simulink model "homeMobileManipulator"  (R2026a)
settings: Solver=ode4  StartTime=0  StopTime=Inf  FixedStep=cfg.rates.plant  MaxStep=cfg.rates.plant  AbsTol=1e-8
PostLoadFcn:
  | hmmSetup;
InitFcn:
  | hmmInitializeRun(bdroot);
values from neighbouring files (symbols this model uses):
  armJointLimits = zeros(numel(idx.arm), 2)    [hmmSetup.m]
  cfg = app.RunCfg    [HomeMobileManipulatorApp.m]    (also in HomeMobileManipulatorExample.m = params.cfg; hmmSetup.m = hmmConfig(); setupParams.m = data.cfg)
undefined symbols (not defined in the file or in its folder): actionQueueInit, actorNameTable, Angle, apertureMap, armPlanInit, Axis, basePlanInit, Custom, Extent, gray, gripperCoupling, invalidRayHits, movableRegistry, objectTargetInit, perceptionStatusInit, placeTargetInit, Position, robotStateInit, Sim3dSensor
libraries: robotmaniplib x20, robotcorelib x18, simulink x9, sim3dcameralib x6, sim3dgroundtruthsensorlib x4, dspmtrx3 x3, slpidlib x3, sim3dlib x3, hdlsllib x2, robotsim3dlib x1
(part 1 of 6)
PreSaveFcn:
  | if exist('hmmCleanBeforeSave', 'file'), hmmCleanBeforeSave(bdroot); end
settings Model: SimulationMode=accelerator  Creator=rvalenti  LastModifiedBy=rvalenti

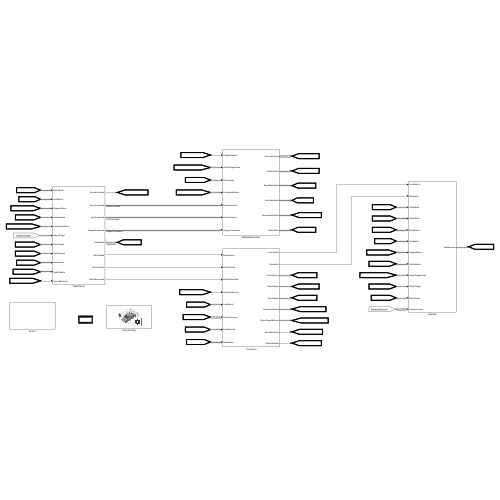
[thumbnail: Simulink's stored preview of the top-level diagram]
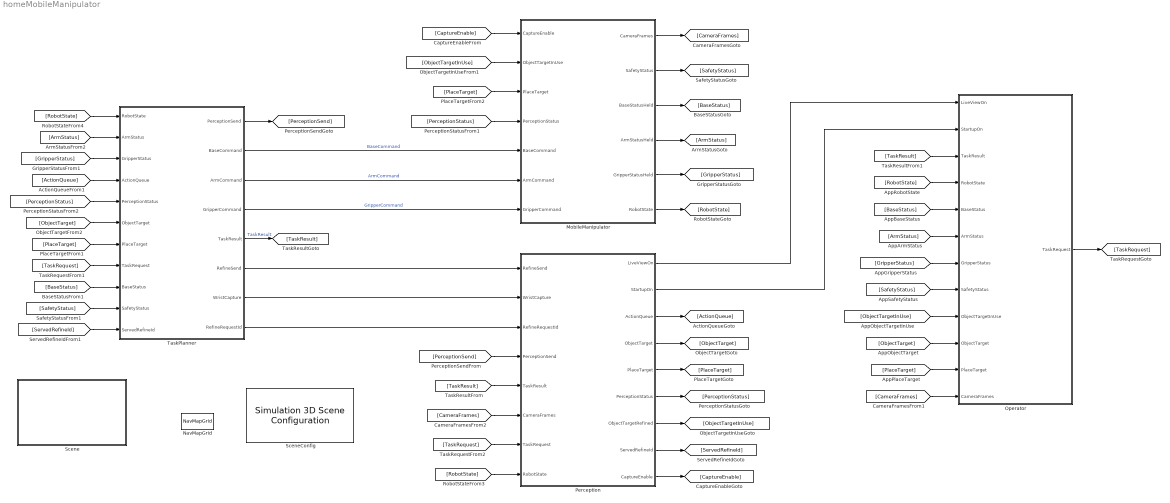
== system homeMobileManipulator ==
  MobileManipulator : Subsystem
  NavMapGrid : DataStoreMemory  DataStoreName=NavMapGrid  InitialValue=navMapGrid  ShowAdditionalParam=off
      settings: DataLoggingMaxPoints=5
  Operator : Subsystem
  Perception : Subsystem
  Scene : Subsystem
  SceneConfig : sim3dlib/Simulation 3D Scene Configuration  Priority=0  ProjectFormat=Default Scenes  SceneDesc=Empty scene  ProjectName=C:\Program Files\MATLAB\R2026a\toolbox\shared\sim3d_projects\automotive_project_windows\UE\WindowsNoEditor\VehicleSimulation.exe  ScenePath=/Game/Maps/EmptyScene  EnableOpenDRIVE=off  vehTagList={'<empty>';'Custom';'Scene Origin';'Sim3dActor1';'Sim3dActor2';'SimulinkVehicle1'}  vehTag=Scene Origin  AttachedCameraRelativeTranslation=[0 0 0]  FreeCameraDefaultInitialTranslation=cfg.view.translation  AttachedCameraRelativeRotation=[0, -15, 0]  FreeCameraDefaultInitialRotation=cfg.view.rotationDeg  ViewpointName=Custom  parentTag=HomeMobileManipulator  FreeCameraInitialTranslation=[0 0 0]  FreeCameraInitialRotation=[0 0 0]  OpVisEn=off  Ts=cfg.rates.scene  EnableWindow=on  EnableRemoteAccess=off  SimulationMode=CoSimulation  SimulateUsing=Interpreted execution  EnableAnimationRecording=off  OverrideDefaultRecording=off  AnimationRecordingFileName=sim3dAnimation.mat  AnimationRecordingInterval=[0 inf]  EnableWeather=off  SunAzimuth=sunAzimuth  SunAltitude=sunAltitude  EnableGeospatialSun=off  Latitude=0  Longitude=0  Date=2023-01-01  Time=10:30:00  GeoTimeZone=-5.0  SunDaylightSaving=off  wind=1  clouds=10  EnableVolumetricClouds=off  CloudCoverage=0  CloudAltitude=6  fog=0  rain=0  RaindropsEffect=off  SnowDensity=0  EnableGeospatial=off  TilesetSource=Earth terrain  UseTrueOrigin=off  OriginHeight=200  OriginLatitude=40.744652  OriginLongitude=-73.988864  MapStyle=Aerial  AdditionalAssetIDs=[]  UseAdvancedSunSky=off  SolarTime=11  TimeZone=-5  Day=21  Month=9  Year=2022  UseDaylightSavingTime=on  DSTStartDay=10  DSTStartMonth=3  DSTEndDay=3  DSTEndMonth=11  DSTSwitchHour=2  sensorTag=MainCamera3  sensorId=3  sensorName=MainCamera3  mountLoc=Origin  offsetFlag=off  tmountOffset=[0, 0, 0]  rmountOffset=[0, 0, 0]  HorizontalResolution=1280  VerticalResolution=720  HorizontalFOV=cfg.view.hfovDeg  mountPoint=[0 0 0]  mountOrientation=[0 0 0]  aMode=5  ID=3  GeoTrigger=Inactive  ViewNameList={'Custom'}  ViewTranslationList={'[0 0 0]'}  ViewRotationList={'[0 0 0]'}
      settings: LibrarySourceBlock=sl3dlib/Simulation 3D/Environment/Simulation 3D Scene Configuration
  TaskPlanner : Subsystem
  wires:
  [TaskRequest] -> TaskPlanner/8(TaskRequest)
  [RobotState] -> TaskPlanner/1(RobotState)
  [ObjectTarget] -> TaskPlanner/6(ObjectTarget)
  [SafetyStatus] -> TaskPlanner/10(SafetyStatus)
  TaskPlanner/5(TaskResult) -> [TaskResult]  "TaskResult"
  [BaseStatus] -> TaskPlanner/9(BaseStatus)
  [ArmStatus] -> TaskPlanner/2(ArmStatus)
  [GripperStatus] -> TaskPlanner/3(GripperStatus)
  [PerceptionStatus] -> TaskPlanner/5(PerceptionStatus)
  [PlaceTarget] -> TaskPlanner/7(PlaceTarget)
  [ActionQueue] -> TaskPlanner/4(ActionQueue)
  [ServedRefineId] -> TaskPlanner/11(ServedRefineId)
  TaskPlanner/2(BaseCommand) -> MobileManipulator/5(BaseCommand)  "BaseCommand"
  TaskPlanner/3(ArmCommand) -> MobileManipulator/6(ArmCommand)  "ArmCommand"
  [ObjectTargetInUse] -> MobileManipulator/2(ObjectTargetInUse)
  [PlaceTarget] -> MobileManipulator/3(PlaceTarget)
  TaskPlanner/4(GripperCommand) -> MobileManipulator/7(GripperCommand)  "GripperCommand"
  MobileManipulator/1(CameraFrames) -> [CameraFrames]
  [PerceptionStatus] -> MobileManipulator/4(PerceptionStatus)
  MobileManipulator/2(SafetyStatus) -> [SafetyStatus]
  MobileManipulator/3(BaseStatusHeld) -> [BaseStatus]
  MobileManipulator/4(ArmStatusHeld) -> [ArmStatus]
  MobileManipulator/5(GripperStatusHeld) -> [GripperStatus]
  MobileManipulator/6(RobotState) -> [RobotState]
  [CameraFrames] -> Perception/6(CameraFrames)
  [TaskRequest] -> Perception/7(TaskRequest)
  [RobotState] -> Perception/8(RobotState)
  Perception/3(ActionQueue) -> [ActionQueue]
  Perception/4(ObjectTarget) -> [ObjectTarget]
  Perception/5(PlaceTarget) -> [PlaceTarget]
  Perception/6(PerceptionStatus) -> [PerceptionStatus]
  TaskPlanner/7(WristCapture) -> Perception/2(WristCapture)
  Perception/9(CaptureEnable) -> [CaptureEnable]
  TaskPlanner/8(RefineRequestId) -> Perception/3(RefineRequestId)
  Perception/7(ObjectTargetRefined) -> [ObjectTargetInUse]
  TaskPlanner/1(PerceptionSend) -> [PerceptionSend]
  TaskPlanner/6(RefineSend) -> Perception/1(RefineSend)
  Perception/8(ServedRefineId) -> [ServedRefineId]
  Operator/1(TaskRequest) -> [TaskRequest]
  [RobotState] -> Operator/4(RobotState)
  [BaseStatus] -> Operator/5(BaseStatus)
  [ArmStatus] -> Operator/6(ArmStatus)
  [GripperStatus] -> Operator/7(GripperStatus)
  [SafetyStatus] -> Operator/8(SafetyStatus)
  [ObjectTargetInUse] -> Operator/9(ObjectTargetInUse)
  [ObjectTarget] -> Operator/10(ObjectTarget)
  [PlaceTarget] -> Operator/11(PlaceTarget)
  [CameraFrames] -> Operator/12(CameraFrames)
  Perception/1(LiveViewOn) -> Operator/1(LiveViewOn)
  Perception/2(StartupOn) -> Operator/2(StartupOn)
  [PerceptionSend] -> Perception/4(PerceptionSend)
  [TaskResult] -> Perception/5(TaskResult)
  [TaskResult] -> Operator/3(TaskResult)
  [CaptureEnable] -> MobileManipulator/1(CaptureEnable)

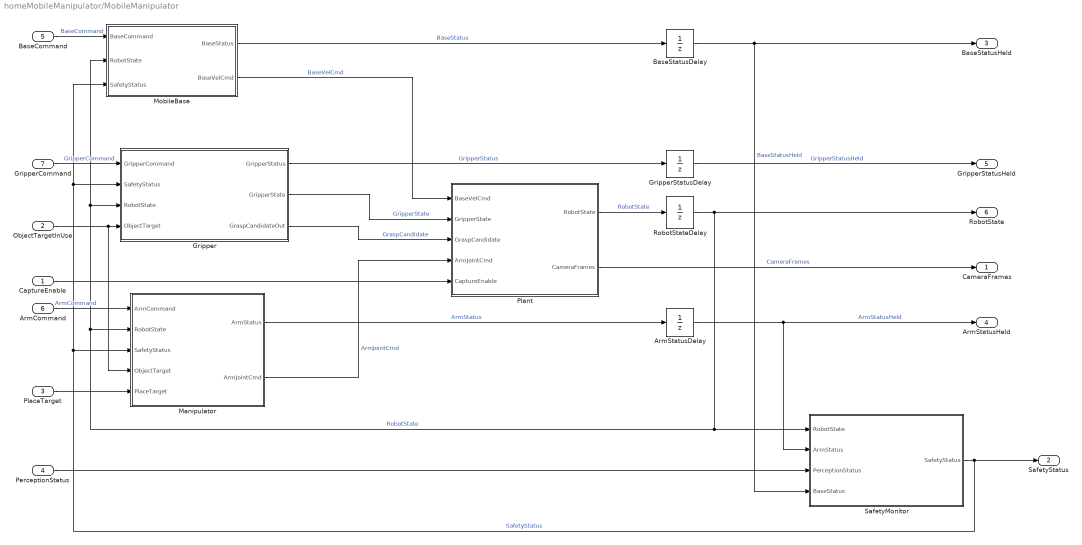
== system homeMobileManipulator/MobileManipulator ==
  CaptureEnable : Inport
  ObjectTargetInUse : Inport  Port=2
  PlaceTarget : Inport  Port=3
  PerceptionStatus : Inport  Port=4
  BaseCommand : Inport  Port=5
  ArmCommand : Inport  Port=6
  GripperCommand : Inport  Port=7
  ArmStatusDelay : UnitDelay  SampleTime=cfg.rates.supervisor
  BaseStatusDelay : UnitDelay  SampleTime=cfg.rates.supervisor
  Gripper : Subsystem
  GripperStatusDelay : UnitDelay  SampleTime=cfg.rates.supervisor
  Manipulator : Subsystem
  MobileBase : Subsystem
  Plant : Subsystem
  RobotStateDelay : UnitDelay  Description=|  InitialCondition=robotStateInit  SampleTime=cfg.rates.plant
      | Breaks the plant-to-supervisor algebraic loop: the supervisors read the robot state and the plant reads their commands, so one of the two has to see the previous step.
      | 
      | THE INITIAL CONDITION IS THE ROBOT'S TRUE STARTING STATE, NOT A ZEROED BUS, AND THAT IS LOAD-BEARING. On the first step every consumer sees this value instead of a measurement. Zeroed, ArmJointPos is the UR5e's fully outstretched pose - tool 1.11 m from arm_mount against a cfg.arm.reach of 0.85 - so SafetyMonitor's reach check fired on sample 0, the e-stop latched, and all four charts sat in their terminal stopped mode for the whole run. hmmSetup builds robotStateInit from cfg.base.initialPose and cfg.arm.stowConfig, the same values the plant's integrators start from, and measures the tool pose off the assembled tree so it cannot drift from the plant's kinematics.
  SafetyMonitor : Subsystem  Description=|  TreatAsAtomicUnit=on  SystemSampleTime=cfg.rates.control
      | Independent limit monitor and the single source of the latched e-stop.
      | 
      | It reads only measured state and reported status - never a chart internal - so a supervisor that has lost track of itself cannot suppress its own e-stop. Every limit is re-evaluated every step; the latch is what makes the result terminal. EStop reaches all four charts (TaskPlanner, BaseSupervisor, ArmSupervisor, GripperSupervisor) through one root Unit Delay, and each has a defined safe terminal mode for it.
      | 
      | ClearanceThreshold is published on the bus rather than assumed, so the value the monitor compared against can be audited against the margin the planner used. hmmSetup/assertConfigInvariants errors at load if the two ever diverge.
  CameraFrames : Outport
  SafetyStatus : Outport  Port=2
  BaseStatusHeld : Outport  Port=3
  ArmStatusHeld : Outport  Port=4
  GripperStatusHeld : Outport  Port=5
  RobotState : Outport  Port=6
  wires:
  BaseStatusDelay/1 -> BaseStatusHeld/1, SafetyMonitor/4(BaseStatus)  "BaseStatusHeld"
  PerceptionStatus/1 -> SafetyMonitor/3(PerceptionStatus)
  Manipulator/2(ArmJointCmd) -> Plant/4(ArmJointCmd)  "ArmJointCmd"
  BaseCommand/1 -> MobileBase/1(BaseCommand)  "BaseCommand"
  GripperCommand/1 -> Gripper/1(GripperCommand)  "GripperCommand"
  ArmCommand/1 -> Manipulator/1(ArmCommand)  "ArmCommand"
  ObjectTargetInUse/1 -> Gripper/4(ObjectTarget), Manipulator/4(ObjectTarget)
  PlaceTarget/1 -> Manipulator/5(PlaceTarget)
  Gripper/1(GripperStatus) -> GripperStatusDelay/1  "GripperStatus"
  Gripper/2(GripperState) -> Plant/2(GripperState)  "GripperState"
  Gripper/3(GraspCandidateOut) -> Plant/3(GraspCandidate)  "GraspCandidate"
  Manipulator/1(ArmStatus) -> ArmStatusDelay/1  "ArmStatus"
  MobileBase/2(BaseVelCmd) -> Plant/1(BaseVelCmd)  "BaseVelCmd"
  MobileBase/1(BaseStatus) -> BaseStatusDelay/1  "BaseStatus"
  CaptureEnable/1 -> Plant/5(CaptureEnable)
  GripperStatusDelay/1 -> GripperStatusHeld/1  "GripperStatusHeld"
  ArmStatusDelay/1 -> ArmStatusHeld/1, SafetyMonitor/2(ArmStatus)  "ArmStatusHeld"
  Plant/1(RobotState) -> RobotStateDelay/1  "RobotState"
  Plant/2(CameraFrames) -> CameraFrames/1  "CameraFrames"
  RobotStateDelay/1 -> RobotState/1, MobileBase/2(RobotState), Gripper/3(RobotState), Manipulator/2(RobotState), SafetyMonitor/1(RobotState)  "RobotState"
  SafetyMonitor/1(SafetyStatus) -> MobileBase/3(SafetyStatus), Gripper/2(SafetyStatus), Manipulator/3(SafetyStatus), SafetyStatus/1  "SafetyStatus"

== system homeMobileManipulator/Operator ==
  LiveViewOn : Inport
  StartupOn : Inport  Port=2
  TaskResult : Inport  Port=3
  RobotState : Inport  Port=4
  BaseStatus : Inport  Port=5
  ArmStatus : Inport  Port=6
  GripperStatus : Inport  Port=7
  SafetyStatus : Inport  Port=8
  ObjectTargetInUse : Inport  Port=9
  ObjectTarget : Inport  Port=10
  PlaceTarget : Inport  Port=11
  CameraFrames : Inport  Port=12
  AppStateTap : MATLAB Function  TreatAsAtomicUnit=on  SystemSampleTime=0.2
  LiveViewTap : MATLAB Function  TreatAsAtomicUnit=on  SystemSampleTime=cfg.rates.perception
  LiveViewTapOpen : Terminator
  TaskRequestSource : MATLAB Function  TreatAsAtomicUnit=on
  TaskRequest : Outport
  wires:
  CameraFrames/1 -> LiveViewTap/1(CameraFrames)
  LiveViewOn/1 -> LiveViewTap/2(LiveViewOn)
  PlaceTarget/1 -> AppStateTap/9(PlaceTarget)
  BaseStatus/1 -> AppStateTap/3(BaseStatus)
  TaskResult/1 -> AppStateTap/2(TaskResult)  "TaskResult"
  StartupOn/1 -> LiveViewTap/3(StartupOn)
  RobotState/1 -> AppStateTap/1(RobotState)
  GripperStatus/1 -> AppStateTap/5(GripperStatus)
  ArmStatus/1 -> AppStateTap/4(ArmStatus)
  SafetyStatus/1 -> AppStateTap/6(SafetyStatus)
  ObjectTargetInUse/1 -> AppStateTap/7(ObjectTargetRefined)
  ObjectTarget/1 -> AppStateTap/8(ObjectTarget)
  TaskRequestSource/1(task) -> TaskRequest/1
  LiveViewTap/1(Fired) -> LiveViewTapOpen/1

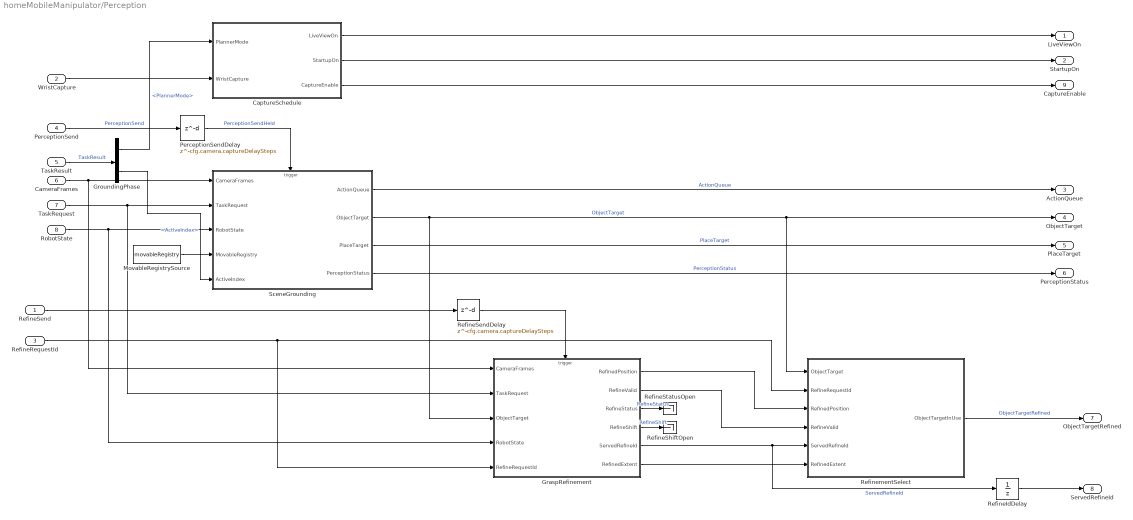
== system homeMobileManipulator/Perception ==
  RefineSend : Inport
  WristCapture : Inport  Port=2
  RefineRequestId : Inport  Port=3
  PerceptionSend : Inport  Port=4
  TaskResult : Inport  Port=5
  CameraFrames : Inport  Port=6
  TaskRequest : Inport  Port=7
  RobotState : Inport  Port=8
  CaptureSchedule : Subsystem
  GraspRefinement : Subsystem
  GroundingPhase : BusSelector  OutputSignals=PlannerMode,ActiveIndex
  MovableRegistrySource : Constant  Value=movableRegistry  OutDataTypeStr=Bus: MovableRegistry  SampleTime=cfg.rates.control
  PerceptionSendDelay : Delay  Description=|  DelayLength=cfg.camera.captureDelaySteps  InitialCondition=0  SampleTime=cfg.rates.supervisor
      | A DELAY OF cfg.camera.captureWindow, NOT A UNIT DELAY, and the length is the whole point. It still breaks the loop from Perception through the planner and back to Perception's trigger, which is why a delay is here at all.
      | 
      | The extra length exists because Plant/CameraRig is now gated on the grounding phase. The planner enters Grounding on a supervisor tick (0.02 s) and the rig captures on a perception tick (0.1 s). With a one-step delay the trigger would fire 0.02 s after the gate opened, before the rig had run, and Perception would read a held frame with Valid = false - or, on a second task, the frame from the first one. Holding the trigger back by three perception periods puts whole capture ticks between the gate opening and Perception looking.
      | 
      | The cost is that every task starts 0.30 s later than it used to. cfg.sup.timeout.ground is 22 s, so the phase has room for it.
      | 
      | See cfg.camera.captureWindow.
  RefineIdDelay : UnitDelay  SampleTime=-1
  RefineSendDelay : Delay  DelayLength=cfg.camera.captureDelaySteps
  RefineShiftOpen : Terminator
  RefineStatusOpen : Terminator
  RefinementSelect : Subsystem
  SceneGrounding : Subsystem
  LiveViewOn : Outport
  StartupOn : Outport  Port=2
  ActionQueue : Outport  Port=3
  ObjectTarget : Outport  Port=4
  PlaceTarget : Outport  Port=5
  PerceptionStatus : Outport  Port=6
  ObjectTargetRefined : Outport  Port=7
  ServedRefineId : Outport  Port=8
  CaptureEnable : Outport  Port=9
  wires:
  PerceptionSend/1 -> PerceptionSendDelay/1  "PerceptionSend"
  GroundingPhase/1 -> CaptureSchedule/1(PlannerMode)  "<PlannerMode>"
  WristCapture/1 -> CaptureSchedule/2(WristCapture)
  CameraFrames/1 -> SceneGrounding/1(CameraFrames), GraspRefinement/1(CameraFrames)
  TaskResult/1 -> GroundingPhase/1  "TaskResult"
  PerceptionSendDelay/1 -> SceneGrounding/Trigger  "PerceptionSendHeld"
  GroundingPhase/2 -> SceneGrounding/5(ActiveIndex)  "<ActiveIndex>"
  MovableRegistrySource/1 -> SceneGrounding/4(MovableRegistry)
  TaskRequest/1 -> SceneGrounding/2(TaskRequest), GraspRefinement/2(TaskRequest)
  RobotState/1 -> SceneGrounding/3(RobotState), GraspRefinement/4(RobotState)
  CaptureSchedule/1(LiveViewOn) -> LiveViewOn/1
  RefineSend/1 -> RefineSendDelay/1
  CaptureSchedule/2(StartupOn) -> StartupOn/1
  CaptureSchedule/3(CaptureEnable) -> CaptureEnable/1
  SceneGrounding/1(ActionQueue) -> ActionQueue/1  "ActionQueue"
  SceneGrounding/2(ObjectTarget) -> ObjectTarget/1, RefinementSelect/1(ObjectTarget), GraspRefinement/3(ObjectTarget)  "ObjectTarget"
  SceneGrounding/3(PlaceTarget) -> PlaceTarget/1  "PlaceTarget"
  SceneGrounding/4(PerceptionStatus) -> PerceptionStatus/1  "PerceptionStatus"
  RefineSendDelay/1 -> GraspRefinement/Trigger
  RefineRequestId/1 -> GraspRefinement/5(RefineRequestId), RefinementSelect/2(RefineRequestId)
  GraspRefinement/1(RefinedPosition) -> RefinementSelect/3(RefinedPosition)
  GraspRefinement/2(RefineValid) -> RefinementSelect/4(RefineValid)
  GraspRefinement/3(RefineStatus) -> RefineStatusOpen/1  "RefineStatus"
  GraspRefinement/4(RefineShift) -> RefineShiftOpen/1  "RefineShift"
  GraspRefinement/5(ServedRefineId) -> RefinementSelect/5(ServedRefineId), RefineIdDelay/1  "ServedRefineId"
  GraspRefinement/6(RefinedExtent) -> RefinementSelect/6(RefinedExtent)
  RefinementSelect/1(ObjectTargetInUse) -> ObjectTargetRefined/1  "ObjectTargetRefined"
  RefineIdDelay/1 -> ServedRefineId/1

== system homeMobileManipulator/Scene ==
  ApartmentShell : sim3dlib/Simulation 3D Actor  Priority=1  ActorName=Sim3dActor1  ParentName=Scene Origin  Operation=Create at setup  InitScriptText=|  SampleTime=-1  Translation=[0 0 0]  Rotation=[0 0 0]  Scale=[1 1 1]  aMode=aMode  ActorTag=Sim3dActor1  ActorType=Sim3dActor  ID=1
      | % Static apartment shell. The mesh is DISCOVERED at init time, never named by
      | % an absolute path in this block, so the model is portable between machines.
      | hmmLoadSceneShell(Actor);
  PropsStatusOpen : Terminator
  SceneProps : sim3dlib/Simulation 3D Actor  Priority=1  ActorName=Sim3dActor2  ParentName=Scene Origin  Operation=Create at setup  InitScriptText=|  SampleTime=-1  Translation=[0 0 0]  Rotation=[0 0 0]  Scale=[1 1 1]  aMode=aMode  ActorTag=Sim3dActor2  ActorType=Sim3dActor  ID=2
      | % Every movable prop the scene manifest lists, spawned as CHILDREN of this
      | % actor. ONE block spawns all of them on purpose: a block per prop would put
      | % the scene's contents into the model, which is the task-specific datum
      | % the design forbids. This actor itself carries no geometry and no transform -
      | % it exists to own the init script and to be the parent, which leaves manifest
      | % coordinates as world coordinates.
      | %
      | % THE PARENT IS NOT DECORATION. Props added at the world root from a block init
      | % script are accepted by the world and never reach the renderer, which is why
      | % this scene had furniture and nothing on it.
      | hmmSpawnProps(World, Actor);
  ShellStatusOpen : Terminator
  wires:
  SceneProps/1 -> PropsStatusOpen/1
  ApartmentShell/1 -> ShellStatusOpen/1

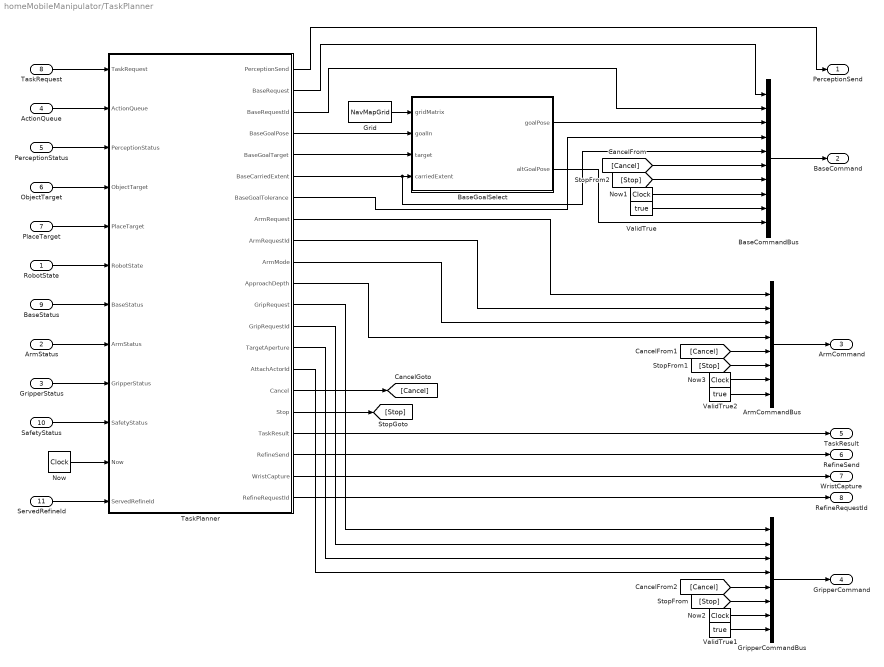
== system homeMobileManipulator/TaskPlanner ==
  RobotState : Inport  OutDataTypeStr=Bus: RobotState
  ArmStatus : Inport  Port=2  OutDataTypeStr=Bus: ArmStatus
  GripperStatus : Inport  Port=3  OutDataTypeStr=Bus: GripperStatus
  ActionQueue : Inport  Port=4  OutDataTypeStr=Bus: ActionQueue
  PerceptionStatus : Inport  Port=5  OutDataTypeStr=Bus: PerceptionStatus
  ObjectTarget : Inport  Port=6  OutDataTypeStr=Bus: ObjectTarget
  PlaceTarget : Inport  Port=7  OutDataTypeStr=Bus: PlaceTarget
  TaskRequest : Inport  Port=8  OutDataTypeStr=Bus: TaskRequest
  BaseStatus : Inport  Port=9  OutDataTypeStr=Bus: BaseStatus
  SafetyStatus : Inport  Port=10  OutDataTypeStr=Bus: SafetyStatus
  ServedRefineId : Inport  Port=11
  ArmCommandBus : BusCreator  Inputs=8  OutDataTypeStr=Bus: ArmCommand
      settings: InheritFromInputs=off
  BaseCommandBus : BusCreator  Inputs=10  OutDataTypeStr=Bus: BaseCommand
      settings: InheritFromInputs=off
  BaseGoalSelect : MATLAB Function  TreatAsAtomicUnit=on
  Grid : DataStoreRead  DataStoreName=NavMapGrid  SampleTime=cfg.rates.supervisor  IndexOptions=Index vector (dialog)  Indices=1  OutputSizes=1
  GripperCommandBus : BusCreator  Inputs=8  OutDataTypeStr=Bus: GripperCommand
      settings: InheritFromInputs=off
  Now{,1..3} (4 alike) : DigitalClock  SampleTime=cfg.rates.supervisor
  TaskPlanner : Stateflow chart  TreatAsAtomicUnit=on
      settings: PortSchema="{\"entries\":[{\"content\":{\"sides\":[{\"content\":{\"connectorIds\":[\"In1\",\"In2\",\"In3\",\"In4\",\"In5\",\"In6\",\"In7\",\"In8\",\"In9\",\"In10\",\"In11\",\"In12\"]},\"type\":\"ConnectorPlacement.EquallySpacedRectSide\",\"uuid\":\"f5e67e83-1d8e-420a-969a-b33278afb01c\"},{\"content\":{\"connectorIds\":[\"Out1\",\"Out2\",\"Out3\",\"Out4\",\"Out5\",\"Out7\",\"Out6\",\"Out8\",\"Out9\",\"Out10\",\"Out11\",\"Out12\",\"Out13\",\"Out14\",\"Out15\",\"Out16\",\"Out17\",\"Out18\",\"Out19\",\"Out20\",\"Out21\"],\"side\":\"RIGHT\"},\"type\":\"ConnectorPlacement.EquallySpacedRectSide\",\"uuid\":\"27a68318-2a47-4f3a-bcd2-e12b0ee86ade\"},{\"content\":{\"side\":\"TOP\"},\"type\":\"ConnectorPlacement.EquallySpacedRectSide\",\"uuid\":\"c7e5a260-d40c-4877-a934-6fb5002bb041\"}]},\"type\":\"ConnectorPlacement.EquallySpacedConnector\",\"uuid\":\"a1ee6b7c-e063-49c8-8f03-48fb3b9dd891\"}],\"packageUris\":[\"http://schema.mathworks.com/mf0/Connector/R2020b\"],\"version\":\"1.0\"}"
  ValidTrue : Constant  Value=true  OutDataTypeStr=boolean
  ValidTrue1 : Constant  Value=true  OutDataTypeStr=boolean
  ValidTrue2 : Constant  Value=true  OutDataTypeStr=boolean
  PerceptionSend : Outport
  BaseCommand : Outport  Port=2  OutDataTypeStr=Bus: BaseCommand
  ArmCommand : Outport  Port=3  OutDataTypeStr=Bus: ArmCommand
  GripperCommand : Outport  Port=4  OutDataTypeStr=Bus: GripperCommand
  TaskResult : Outport  Port=5  OutDataTypeStr=Bus: TaskResult
  RefineSend : Outport  Port=6
  WristCapture : Outport  Port=7
  RefineRequestId : Outport  Port=8
  wires:
  TaskPlanner/19(RefineSend) -> RefineSend/1
  TaskRequest/1 -> TaskPlanner/1(TaskRequest)
  BaseStatus/1 -> TaskPlanner/7(BaseStatus)
  PerceptionStatus/1 -> TaskPlanner/3(PerceptionStatus)
  ActionQueue/1 -> TaskPlanner/2(ActionQueue)
  ObjectTarget/1 -> TaskPlanner/4(ObjectTarget)
  Grid/1 -> BaseGoalSelect/1(gridMatrix)
  PlaceTarget/1 -> TaskPlanner/5(PlaceTarget)
  RobotState/1 -> TaskPlanner/6(RobotState)
  ArmStatus/1 -> TaskPlanner/8(ArmStatus)
  TaskPlanner/6(BaseGoalTolerance) -> BaseCommandBus/4
  GripperStatus/1 -> TaskPlanner/9(GripperStatus)
  TaskPlanner/15(AttachActorId) -> GripperCommandBus/4
  ServedRefineId/1 -> TaskPlanner/12(ServedRefineId)
  SafetyStatus/1 -> TaskPlanner/10(SafetyStatus)
  Now2/1 -> GripperCommandBus/7
  TaskPlanner/13(GripRequestId) -> GripperCommandBus/2
  Now/1 -> TaskPlanner/11(Now)
  TaskPlanner/3(BaseRequestId) -> BaseCommandBus/2
  TaskPlanner/2(BaseRequest) -> BaseCommandBus/1
  TaskPlanner/1(PerceptionSend) -> PerceptionSend/1
  GripperCommandBus/1 -> GripperCommand/1
  TaskPlanner/4(BaseGoalPose) -> BaseGoalSelect/2(goalIn)
  TaskPlanner/14(TargetAperture) -> GripperCommandBus/3
  TaskPlanner/5(BaseGoalTarget) -> BaseGoalSelect/3(target)
  Now3/1 -> ArmCommandBus/7
  TaskPlanner/7(BaseCarriedExtent) -> BaseCommandBus/5, BaseGoalSelect/4(carriedExtent)
  TaskPlanner/8(ArmRequest) -> ArmCommandBus/1
  TaskPlanner/9(ArmRequestId) -> ArmCommandBus/2
  Now1/1 -> BaseCommandBus/8
  TaskPlanner/10(ArmMode) -> ArmCommandBus/3
  TaskPlanner/11(ApproachDepth) -> ArmCommandBus/4
  TaskPlanner/12(GripRequest) -> GripperCommandBus/1
  TaskPlanner/18(TaskResult) -> TaskResult/1
  TaskPlanner/20(WristCapture) -> WristCapture/1
  TaskPlanner/21(RefineRequestId) -> RefineRequestId/1
  ValidTrue2/1 -> ArmCommandBus/8
  ValidTrue1/1 -> GripperCommandBus/8
  BaseGoalSelect/1(goalPose) -> BaseCommandBus/3
  BaseGoalSelect/2(altGoalPose) -> BaseCommandBus/10
  ValidTrue/1 -> BaseCommandBus/9
  ArmCommandBus/1 -> ArmCommand/1
  BaseCommandBus/1 -> BaseCommand/1
  TaskPlanner/16(Cancel) -> [Cancel]
  [Cancel] -> BaseCommandBus/6
  [Cancel] -> ArmCommandBus/5
  [Cancel] -> GripperCommandBus/5
  TaskPlanner/17(Stop) -> [Stop]
  [Stop] -> GripperCommandBus/6
  [Stop] -> ArmCommandBus/6
  [Stop] -> BaseCommandBus/7

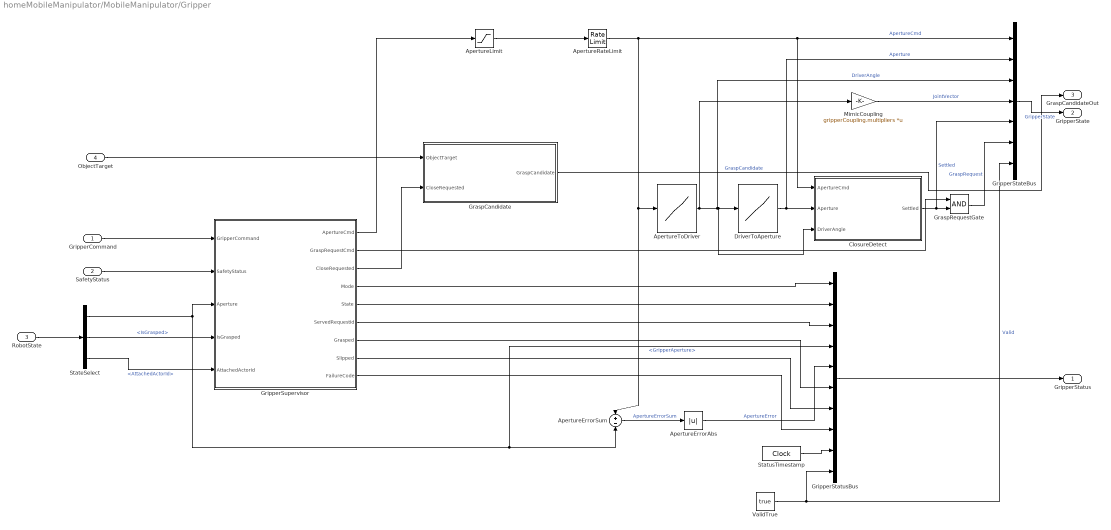
== system homeMobileManipulator/MobileManipulator/Gripper ==
  GripperCommand : Inport  OutDataTypeStr=Bus: GripperCommand
  SafetyStatus : Inport  Port=2  OutDataTypeStr=Bus: SafetyStatus
  RobotState : Inport  Port=3  OutDataTypeStr=Bus: RobotState
  ObjectTarget : Inport  Port=4  OutDataTypeStr=Bus: ObjectTarget
  ApertureErrorAbs : Abs
  ApertureErrorSum : Sum  Inputs=+-
  ApertureLimit : Saturate  UpperLimit=apertureMap.apertureBreakpoints(end)  LowerLimit=apertureMap.apertureBreakpoints(1)
  ApertureRateLimit : RateLimiter  RisingSlewLimit=cfg.gripper.apertureRateMax  FallingSlewLimit=-cfg.gripper.apertureRateMax
  ApertureToDriver : Lookup_n-D  NumberOfTableDimensions=1  BreakpointsForDimension1=apertureMap.apertureBreakpoints  Table=apertureMap.driverTable  ExtrapMethod=Clip  InternalRulePriority=Speed  RndMeth=Simplest
  ClosureDetect : Subsystem
  DriverToAperture : Lookup_n-D  NumberOfTableDimensions=1  BreakpointsForDimension1=apertureMap.driverBreakpoints  Table=apertureMap.apertureTable  ExtrapMethod=Clip  InternalRulePriority=Speed  RndMeth=Simplest
  GraspCandidate : Subsystem  Description=|  TreatAsAtomicUnit=on  SystemSampleTime=cfg.rates.supervisor
      | Assembles the GraspCandidate bus the Plant's attach logic consumes.
      | 
      | PERIODIC ATOMIC AT THE SUPERVISOR RATE, DELIBERATELY. GraspCandidate is read by a
      | Stateflow chart, so Simulink makes the bus NONVIRTUAL, and every signal feeding a
      | nonvirtual Bus Creator must share one sample time. The candidate mixes perception-rate
      | fields (0.1 s) with supervisor-rate ones, which is exactly what that rule forbids, so
      | the rate is declared here once instead of on each block inside: an atomic subsystem
      | with a periodic sample time runs everything it contains at that rate. The three blocks
      | that used to carry cfg.rates.perception now inherit it. Nothing is lost - re-evaluating
      | a held perception value five times as often returns the same value - and the gain is
      | that the candidate is published on the same clock as the gripper it belongs to.
  GraspRequestGate : Logic  AllPortsSameDT=off  OutDataTypeStr=boolean
  GripperStateBus : BusCreator  Inputs=7  OutDataTypeStr=Bus: GripperState
      settings: InheritFromInputs=off
  GripperStatusBus : BusCreator  Inputs=10  OutDataTypeStr=Bus: GripperStatus
      settings: InheritFromInputs=off
  GripperSupervisor : Stateflow chart  TreatAsAtomicUnit=on
  MimicCoupling : Gain  Gain=gripperCoupling.multipliers  Multiplication=Matrix(K*u)
  StateSelect : BusSelector  OutputSignals=GripperAperture,IsGrasped,AttachedActorId
  StatusTimestamp : DigitalClock  SampleTime=cfg.rates.supervisor
  ValidTrue : Constant  Value=true  OutDataTypeStr=boolean
  GripperStatus : Outport  OutDataTypeStr=Bus: GripperStatus
  GripperState : Outport  Port=2  OutDataTypeStr=Bus: GripperState
  GraspCandidateOut : Outport  Port=3  OutDataTypeStr=Bus: GraspCandidate
  wires:
  GripperStateBus/1 -> GripperState/1  "GripperState"
  GraspRequestGate/1 -> GripperStateBus/6  "GraspRequest"
  GripperStatusBus/1 -> GripperStatus/1
  ClosureDetect/1(Settled) -> GripperStateBus/5, GraspRequestGate/2  "Settled"
  MimicCoupling/1 -> GripperStateBus/4  "JointVector"
  ApertureErrorAbs/1 -> GripperStatusBus/5  "ApertureError"
  DriverToAperture/1 -> GripperStateBus/2, ClosureDetect/2(Aperture)  "Aperture"
  ApertureErrorSum/1 -> ApertureErrorAbs/1  "ApertureErrorSum"
  GraspCandidate/1(GraspCandidate) -> GraspCandidateOut/1  "GraspCandidate"
  GripperSupervisor/9(FailureCode) -> GripperStatusBus/8
  GripperSupervisor/8(Slipped) -> GripperStatusBus/7
  GripperSupervisor/7(Grasped) -> GripperStatusBus/6
  GripperSupervisor/6(ServedRequestId) -> GripperStatusBus/3
  GripperSupervisor/5(State) -> GripperStatusBus/2
  GripperSupervisor/4(Mode) -> GripperStatusBus/1
  GripperSupervisor/3(CloseRequested) -> GraspCandidate/2(CloseRequested)
  GripperSupervisor/2(GraspRequestCmd) -> GraspRequestGate/1
  GripperSupervisor/1(ApertureCmd) -> ApertureLimit/1
  ApertureToDriver/1 -> DriverToAperture/1, ClosureDetect/3(DriverAngle), GripperStateBus/3, MimicCoupling/1  "DriverAngle"
  RobotState/1 -> StateSelect/1
  StatusTimestamp/1 -> GripperStatusBus/9
  StateSelect/1 -> GripperStatusBus/4, ApertureErrorSum/2, GripperSupervisor/3(Aperture)  "<GripperAperture>"
  GripperCommand/1 -> GripperSupervisor/1(GripperCommand)
  ApertureLimit/1 -> ApertureRateLimit/1
  StateSelect/2 -> GripperSupervisor/4(IsGrasped)  "<IsGrasped>"
  ApertureRateLimit/1 -> ApertureErrorSum/1, ApertureToDriver/1, GripperStateBus/1, ClosureDetect/1(ApertureCmd)  "ApertureCmd"
  StateSelect/3 -> GripperSupervisor/5(AttachedActorId)  "<AttachedActorId>"
  SafetyStatus/1 -> GripperSupervisor/2(SafetyStatus)
  ObjectTarget/1 -> GraspCandidate/1(ObjectTarget)
  ValidTrue/1 -> GripperStatusBus/10, GripperStateBus/7  "Valid"

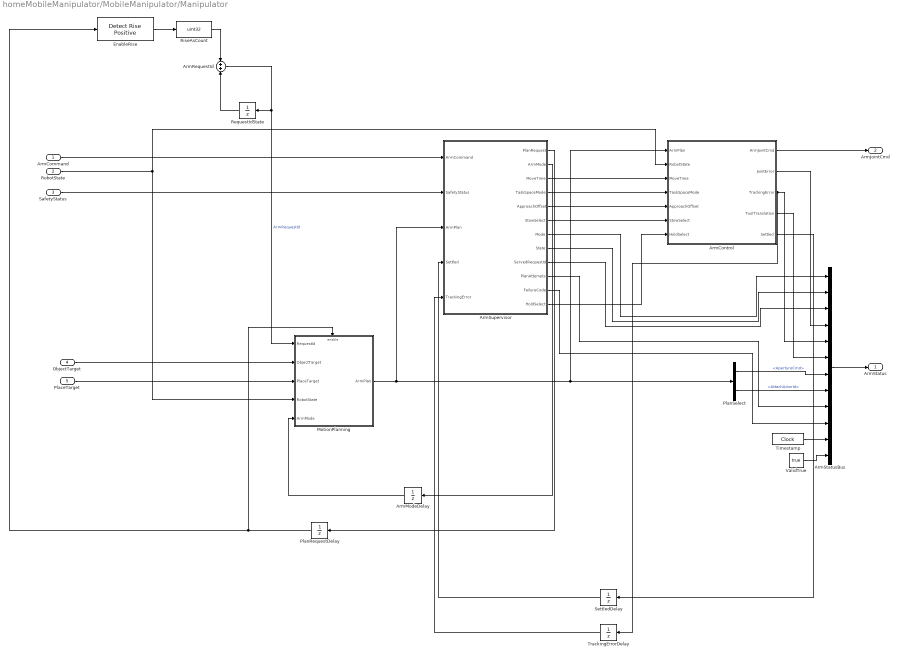
== system homeMobileManipulator/MobileManipulator/Manipulator ==
  ArmCommand : Inport  OutDataTypeStr=Bus: ArmCommand
  RobotState : Inport  Port=2  OutDataTypeStr=Bus: RobotState
  SafetyStatus : Inport  Port=3  OutDataTypeStr=Bus: SafetyStatus
  ObjectTarget : Inport  Port=4  OutDataTypeStr=Bus: ObjectTarget
  PlaceTarget : Inport  Port=5  OutDataTypeStr=Bus: PlaceTarget
  ArmControl : Subsystem
  ArmModeDelay : UnitDelay  InitialCondition=cfg.plan.ARM_MODE_PICK  SampleTime=cfg.rates.supervisor
  ArmRequestId : Sum  OutDataTypeStr=uint32
  ArmStatusBus : BusCreator  Inputs=12  OutDataTypeStr=Bus: ArmStatus
      settings: InheritFromInputs=off
  ArmSupervisor : Stateflow chart  TreatAsAtomicUnit=on
  EnableRise : hdlsllib/Logic and Bit Operations/Detect Rise Positive  vinit=0  OutDataTypeStr=boolean
  MotionPlanning : Subsystem
  PlanRequestDelay : UnitDelay  InitialCondition=false  SampleTime=cfg.rates.supervisor
  PlanSelect : BusSelector  OutputSignals=ApertureCmd,AttachActorId
  RequestIdState : UnitDelay  SampleTime=-1
  RiseAsCount : DataTypeConversion  OutDataTypeStr=uint32  SaturateOnIntegerOverflow=off  RndMeth=Floor
  SettledDelay : UnitDelay  InitialCondition=false  SampleTime=cfg.rates.supervisor
  Timestamp : DigitalClock  SampleTime=cfg.rates.supervisor
  TrackingErrorDelay : UnitDelay  SampleTime=cfg.rates.supervisor
  ValidTrue : Constant  Value=true  OutDataTypeStr=boolean
  ArmStatus : Outport  OutDataTypeStr=Bus: ArmStatus
  ArmJointCmd : Outport  Port=2
  wires:
  ArmStatusBus/1 -> ArmStatus/1
  ValidTrue/1 -> ArmStatusBus/12
  PlanSelect/2 -> ArmStatusBus/8  "<AttachActorId>"
  PlanSelect/1 -> ArmStatusBus/7  "<ApertureCmd>"
  ArmControl/3(TrackingError) -> ArmStatusBus/5, TrackingErrorDelay/1
  ArmControl/1(ArmJointCmd) -> ArmJointCmd/1
  SettledDelay/1 -> ArmSupervisor/4(Settled)
  ArmSupervisor/12(HoldSelect) -> ArmControl/7(HoldSelect)
  Timestamp/1 -> ArmStatusBus/11
  ArmSupervisor/11(FailureCode) -> ArmStatusBus/10
  ArmSupervisor/9(ServedRequestId) -> ArmStatusBus/3
  ArmSupervisor/8(State) -> ArmStatusBus/2
  ArmSupervisor/7(Mode) -> ArmStatusBus/1
  TrackingErrorDelay/1 -> ArmSupervisor/5(TrackingError)
  ArmSupervisor/5(ApproachOffset) -> ArmControl/5(ApproachOffset)
  ArmSupervisor/4(TaskSpaceMode) -> ArmControl/4(TaskSpaceMode)
  ArmSupervisor/3(MoveTime) -> ArmControl/3(MoveTime)
  ArmSupervisor/2(ArmMode) -> ArmModeDelay/1
  ArmSupervisor/1(PlanRequest) -> PlanRequestDelay/1
  ArmControl/5(Settled) -> SettledDelay/1
  SafetyStatus/1 -> ArmSupervisor/2(SafetyStatus)
  ArmControl/4(ToolTranslation) -> ArmStatusBus/6
  ArmCommand/1 -> ArmSupervisor/1(ArmCommand)
  PlanRequestDelay/1 -> EnableRise/1, MotionPlanning/Enable
  ArmModeDelay/1 -> MotionPlanning/5(ArmMode)
  RobotState/1 -> MotionPlanning/4(RobotState), ArmControl/2(RobotState)
  ArmControl/2(JointError) -> ArmStatusBus/4
  ObjectTarget/1 -> MotionPlanning/2(ObjectTarget)
  PlaceTarget/1 -> MotionPlanning/3(PlaceTarget)
  ArmRequestId/1 -> RequestIdState/1, MotionPlanning/1(RequestId)  "ArmRequestId"
  RiseAsCount/1 -> ArmRequestId/1
  RequestIdState/1 -> ArmRequestId/2
  EnableRise/1 -> RiseAsCount/1
  ArmSupervisor/6(StowSelect) -> ArmControl/6(StowSelect)
  MotionPlanning/1(ArmPlan) -> PlanSelect/1, ArmControl/1(ArmPlan), ArmSupervisor/3(ArmPlan)
  ArmSupervisor/10(PlanAttempts) -> ArmStatusBus/9

== system homeMobileManipulator/MobileManipulator/MobileBase ==
  BaseCommand : Inport  OutDataTypeStr=Bus: BaseCommand  PortDimensions=3
  RobotState : Inport  Port=2  OutDataTypeStr=Bus: RobotState
  SafetyStatus : Inport  Port=3  OutDataTypeStr=Bus: SafetyStatus  PortDimensions=3
  BaseAccelLimit : RateLimiter  RisingSlewLimit=cfg.base.slewMargin * [cfg.base.axMax; cfg.base.ayMax; cfg.base.alphaMax]  FallingSlewLimit=-cfg.base.slewMargin * [cfg.base.axMax; cfg.base.ayMax; cfg.base.alphaMax]  SampleTimeMode=inherited  InitialCondition=zeros(3,1)
  BaseStatusBus : BusCreator  Inputs=12  OutDataTypeStr=Bus: BaseStatus
      settings: InheritFromInputs=off
  BaseSupervisor : Stateflow chart  TreatAsAtomicUnit=on
  CommandSelect : BusSelector  OutputSignals=GoalPose,GoalTolerance,CarriedExtent,AltGoalPose
  FollowEnableDelay : UnitDelay  InitialCondition=false  SampleTime=cfg.rates.supervisor
  FollowTimeDelay : UnitDelay  SampleTime=cfg.rates.supervisor
  PathFollowing : Subsystem
  PathPlanning : Subsystem
  PlanGoalSelect : BusSelector  OutputSignals=GoalPose
  PlanRequestDelay : UnitDelay  InitialCondition=false  SampleTime=cfg.rates.supervisor
  Timestamp : DigitalClock  SampleTime=cfg.rates.supervisor
  ValidTrue : Constant  Value=true  OutDataTypeStr=boolean
  BaseStatus : Outport  OutDataTypeStr=Bus: BaseStatus
  BaseVelCmd : Outport  Port=2
  wires:
  ValidTrue/1 -> BaseStatusBus/12
  SafetyStatus/1 -> BaseSupervisor/2(SafetyStatus)
  Timestamp/1 -> BaseStatusBus/11
  FollowEnableDelay/1 -> PathFollowing/Enable
  PathFollowing/4(CrossTrackError) -> BaseSupervisor/5(CrossTrackError), BaseStatusBus/6
  PathFollowing/3(HeadingError) -> BaseStatusBus/5
  PathFollowing/1(BaseVelCmd) -> BaseAccelLimit/1
  PlanRequestDelay/1 -> PathPlanning/Trigger
  PlanGoalSelect/1 -> PathFollowing/2(GoalPose)  "<GoalPose>"
  BaseAccelLimit/1 -> BaseVelCmd/1
  PathPlanning/1(BasePlan) -> PlanGoalSelect/1, PathFollowing/4(BasePlan), BaseSupervisor/3(BasePlan)
  PathFollowing/2(DistanceToGoal) -> BaseStatusBus/4
  CommandSelect/3 -> PathPlanning/3(CarriedExtent)  "<CarriedExtent>"
  PathFollowing/5(AtGoal) -> BaseSupervisor/4(AtGoal)
  BaseStatusBus/1 -> BaseStatus/1
  CommandSelect/4 -> PathPlanning/4(AltGoalPose)  "<AltGoalPose>"
  CommandSelect/2 -> PathFollowing/3(GoalTolerance)  "<GoalTolerance>"
  FollowTimeDelay/1 -> PathFollowing/5(FollowTime)
  RobotState/1 -> PathPlanning/1(RobotState), PathFollowing/1(RobotState), BaseSupervisor/6(RobotState)
  CommandSelect/1 -> PathPlanning/2(GoalPose)  "<GoalPose>"
  BaseCommand/1 -> CommandSelect/1, BaseSupervisor/1(BaseCommand)
  BaseSupervisor/8(PlanRequest) -> PlanRequestDelay/1
  BaseSupervisor/9(FollowEnable) -> FollowEnableDelay/1
  BaseSupervisor/10(FollowTime) -> FollowTimeDelay/1
  BaseSupervisor/1(Mode) -> BaseStatusBus/1
  BaseSupervisor/2(State) -> BaseStatusBus/2
  BaseSupervisor/3(ServedRequestId) -> BaseStatusBus/3
  BaseSupervisor/6(PlanAttempts) -> BaseStatusBus/9
  BaseSupervisor/7(FailureCode) -> BaseStatusBus/10
  BaseSupervisor/5(ReplanRequest) -> BaseStatusBus/8
  BaseSupervisor/4(Stalled) -> BaseStatusBus/7

== system homeMobileManipulator/MobileManipulator/Plant ==
  BaseVelCmd : Inport
  GripperState : Inport  Port=2  OutDataTypeStr=Bus: GripperState
  GraspCandidate : Inport  Port=3  OutDataTypeStr=Bus: GraspCandidate
  ArmJointCmd : Inport  Port=4
  CaptureEnable : Inport  Port=5
  ArmKinematics : Subsystem  Description=Arm plant: a velocity-limited first-order joint servo (command -> position limit -> 1/cfg.arm.jointTimeConst -> cfg.arm.jointVelMax saturation -> integrator). Deliberately NOT a Joint Space Motion Model: every JSMM motion type is a second-order response (PD, computed torque, or independent joints by damping ratio/natural frequency) with no velocity or position saturation, and the joint velocity limit is the defining physical constraint the planners respect and SafetyMonitor checks. JSMM is used where it fits, as the reference shaper in ArmControl/JointSpaceTrack. Checked 2026-10-08.
  BaseKinematics : Subsystem
  CameraRig : Subsystem  Description=|
      | GATHERED ONCE PER TASK, NOT EVERY TENTH OF A SECOND. This subsystem is ENABLED on TaskResult.PlannerMode == cfg.sup.pl.GROUND, so the five Simulation 3D Cameras and the four Ray Tracers run only while the planner is grounding an instruction.
      | 
      | It used to run unconditionally at cfg.rates.perception - 400 times over the 40 s reference run - and be READ once. Perception is a triggered subsystem, one grounding call yields the whole action queue, and Plant/CameraFrames has exactly one destination. 3,686,400 ray casts were made and 9,216 read.
      | 
      | CameraFrames is held when disabled, so the last frame and its CaptureTime both freeze. That is deliberate: a frozen timestamp is what lets hmmGroundingService and hmmReconstructTargets test a real age against cfg.safety.staleTimeout instead of trusting a clock that kept running.
      | 
      | See cfg.camera.captureWindow.
  ChaseCamera : Subsystem  Description=A view that follows the robot, beside the full one: a Simulation 3D Camera posed from chassis_link by cfg.view.chase.offset, shown in a Video Viewer. Display only - nothing reads it.
  ChaseViewOn : MATLAB Function  TreatAsAtomicUnit=on  SystemSampleTime=cfg.rates.scene
  GraspCaptureGate : Subsystem
  GripperStateSelect : BusSelector  OutputSignals=JointVector,Aperture,DriverAngle,GraspRequest
  RobotActor : Subsystem  Description=|
      | Sim3D bridge for the one authoritative 15-DOF rigidBodyTree.
      | 
      | The actor is posed ONLY by the 15-element Config vector: Simulation 3D Robot
      | is configured with inpTransEnbVal off, so it has no actor-root Translation or
      | Rotation inputs at all. There is therefore no way to move the base separately
      | from the arm, and the artefact where a base translates before its
      | arm follows is structurally unreachable rather than merely avoided.
      | 
      | AttachedActorId reports what the ENGINE has attached, not what the capture gate
      | asked for: the gate's TargetActorId passes through only while IsTargetGrasped
      | is true, and reads cfg.actor.noneId otherwise. Resolving it here rather than in
      | StateReport is deliberate - both signals exist natively at this level, so no
      | feedback path around the Sim3D block is needed to answer the question.
  StateReport : Subsystem  Description=|  TreatAsAtomicUnit=on  SystemSampleTime=cfg.rates.plant
      | Pure interface assembler: one Bus Creator, no logic.
      | 
      | Inport order is the RobotState element order, so the wiring is checkable by
      | reading down the port list rather than by tracing lines. Timestamp and Valid
      | are produced here because they describe THIS report and have no upstream source.
      | 
      | This subsystem holds 17 blocks, above the ~15 guideline. Thirteen of them are
      | inports and the count is irreducible: a 15-element interface bus needs 15
      | sources at one level, and nesting the bus to shrink the port list would change
      | the interface contract handed to the perception and supervisory stages.
  ToolKinematics : Subsystem
  RobotState : Outport  OutDataTypeStr=Bus: RobotState
  CameraFrames : Outport  Port=2
  wires:
  CameraRig/1(CameraFrames) -> CameraFrames/1
  RobotActor/5(AttachedActorId) -> StateReport/12(AttachedActorId)  "AttachedActorId"
  RobotActor/3(ActorRotation) -> StateReport/11(ActorRotation)  "ActorRotation"
  RobotActor/4(IsGrasped) -> StateReport/13(IsGrasped)  "IsGrasped"
  GraspCaptureGate/3(TargetActorName) -> RobotActor/6(TargetActorName)  "TargetActorName"
  CaptureEnable/1 -> CameraRig/Enable
  GraspCaptureGate/1(TargetActorId) -> RobotActor/4(TargetActorId)  "TargetActorId"
  ArmKinematics/2(ArmJointVel) -> StateReport/5(ArmJointVel)  "ArmJointVel"
  BaseKinematics/3(WheelSpeeds) -> StateReport/3(WheelSpeeds)  "WheelSpeeds"
  BaseKinematics/1(BasePose) -> RobotActor/3(BasePose), StateReport/1(BasePose)  "BasePose"
  BaseKinematics/2(BaseTwist) -> StateReport/2(BaseTwist)  "BaseTwist"
  ToolKinematics/3(GraspFramePos) -> GraspCaptureGate/3(GraspFramePos)  "GraspFramePos"
  RobotActor/1(RobotConfig) -> CameraRig/1(RobotConfig), ChaseCamera/1(RobotConfig), ToolKinematics/1(RobotConfig)  "RobotConfig"
  RobotActor/2(ActorTranslation) -> StateReport/10(ActorTranslation)  "ActorTranslation"
  ToolKinematics/2(ToolRotation) -> StateReport/9(ToolRotation)  "ToolRotation"
  GraspCaptureGate/2(ActivateGrasp) -> RobotActor/5(ActivateGrasp)  "ActivateGrasp"
  ToolKinematics/1(ToolTranslation) -> StateReport/8(ToolTranslation)  "ToolTranslation"
  GripperStateSelect/4 -> GraspCaptureGate/1(GraspRequest)  "<GraspRequest>"
  ArmKinematics/1(ArmJointPos) -> RobotActor/2(ArmJointPos), StateReport/4(ArmJointPos)  "ArmJointPos"
  GraspCandidate/1 -> GraspCaptureGate/4(GraspCandidate)
  GripperStateSelect/3 -> StateReport/7(GripperDriverAngle)  "<DriverAngle>"
  GripperStateSelect/2 -> StateReport/6(GripperAperture), GraspCaptureGate/2(AchievedAperture)  "<Aperture>"
  ArmJointCmd/1 -> ArmKinematics/1(ArmJointCmd)
  StateReport/1(RobotState) -> RobotState/1
  BaseVelCmd/1 -> BaseKinematics/1(BaseVelCmd)
  GripperStateSelect/1 -> RobotActor/1(GripperJointVector)  "<JointVector>"
  GripperState/1 -> GripperStateSelect/1
  ChaseViewOn/1(on) -> ChaseCamera/Enable

== system homeMobileManipulator/MobileManipulator/SafetyMonitor ==
  RobotState : Inport  OutDataTypeStr=Bus: RobotState
  ArmStatus : Inport  Port=2  OutDataTypeStr=Bus: ArmStatus
  PerceptionStatus : Inport  Port=3  OutDataTypeStr=Bus: PerceptionStatus
  BaseStatus : Inport  Port=4  OutDataTypeStr=Bus: BaseStatus
  BaseLimitChecks : Subsystem
  CausePriority : Subsystem  Description=|
      | Lowest active cfg.sup.cause code, and whether anything is raised at all.
      | 
      | A Switch replaces each raised flag with its cause code and each clear flag with 255, and one MinMax configured for a single input reduces over the vector. Lowest-code-wins gives a fixed, documented priority order without a chain of nested Switches, and the code vector is built from the NAMED cfg.sup.cause fields rather than from 1:nCauses, so renumbering the causes in hmmConfig moves the priorities with them instead of silently relabelling them.
      | 
      | When nothing is raised the reduction returns 255, which is why the result is tested against nCauses rather than against zero, and mapped back to cause.NONE - 255 is not a cause, it is the absence of one.
  EStopLatch : Subsystem  Description=|
      | EStop = AnyFault OR EStop[k-1]. Once true it stays true for the whole run.
      | 
      | LatchedCause holds the FIRST cause, and the Switch that selects it is controlled by the DELAYED EStop, not the live one. On the step the latch closes, the live EStop is already true, so a Switch driven by it would select the held value - which is still cause.NONE - and the run would report a latched e-stop with no cause. Driving the Switch from EStop[k-1] admits the live cause on exactly the latching step and holds it from then on.
      | 
      | Both Unit Delays inherit their sample time rather than naming one, so the latch always runs at the same rate as the fault detection feeding it. A latch sampled slower than its input can step straight over a one-step fault pulse.
  FlagVector : Mux  Inputs=9
  JointChecks : Subsystem  Description=|
      | Arm joint position, speed and acceleration against armJointLimits, cfg.arm.jointVelMax and cfg.arm.jointAccMax.
      | 
      | The position test is two-sided (q < lower OR q > upper) even though this robot's limits happen to be symmetric, so abs(q) > upper would give the same answer today. Relying on that symmetry would make the check silently miss every lower-limit violation the day the URDF is swapped for a robot with asymmetric joints, and nothing in the model would report it.
      | 
      | Each of the three tests reduces its 6-element boolean result to one flag with a single OR block configured for one input, which reduces over the elements.
  Now : DigitalClock  SampleTime=cfg.rates.control
  Now1 : DigitalClock  SampleTime=cfg.rates.control
  SafetyStatusBus : BusCreator  Inputs=13  OutDataTypeStr=Bus: SafetyStatus
      settings: InheritFromInputs=off
  StalenessCheck : Subsystem  Description=|
      | Age of the measured state, the subordinate statuses and the grounding provider.
      | 
      | HONEST LIMITATION. In the delivered single-rate, always-enabled configuration StaleState and StalePlan cannot fire: RobotState, BaseStatus and ArmStatus are each stamped by a Digital Clock inside a subsystem that runs every step, so their age is identically zero. They are built correctly and left in place because moving any of those producers behind an enable, onto a slower rate or into a model reference makes them live immediately, and a monitor that would have to be extended at that point is a monitor nobody extends. StaleProvider IS live: Perception is triggered, so its timestamp freezes between requests.
      | 
      | All four tests share one gated age test, so none of them can drift from the others. See StateStale for why the gate is not optional.
  StateSelect : BusSelector  OutputSignals=ArmJointPos,ArmJointVel,BaseTwist,ToolTranslation
  ValidTrue : Constant  Value=true  OutDataTypeStr=boolean
  WorkspaceCheck : Subsystem
  SafetyStatus : Outport  OutDataTypeStr=Bus: SafetyStatus
  wires:
  SafetyStatusBus/1 -> SafetyStatus/1
  EStopLatch/2(LatchedCause) -> SafetyStatusBus/2
  EStopLatch/1(EStop) -> SafetyStatusBus/1
  FlagVector/1 -> CausePriority/1(Flags)  "FlagVector"
  StalenessCheck/3(StaleProvider) -> FlagVector/9, SafetyStatusBus/11
  StalenessCheck/1(StaleState) -> FlagVector/7, SafetyStatusBus/9
  BaseLimitChecks/2(BaseAccel) -> FlagVector/6, SafetyStatusBus/8
  BaseLimitChecks/1(BaseVel) -> FlagVector/5, SafetyStatusBus/7
  JointChecks/2(JointVel) -> FlagVector/2, SafetyStatusBus/4
  JointChecks/3(JointAccel) -> SafetyStatusBus/5, FlagVector/3
  JointChecks/1(JointLimit) -> FlagVector/1, SafetyStatusBus/3
  Now1/1 -> SafetyStatusBus/12
  Now/1 -> StalenessCheck/5(Now)
  PerceptionStatus/1 -> StalenessCheck/4(PerceptionStatus)
  ArmStatus/1 -> StalenessCheck/3(ArmStatus)
  BaseStatus/1 -> StalenessCheck/2(BaseStatus)
  CausePriority/2(AnyFault) -> EStopLatch/1(AnyFault)
  StateSelect/4 -> WorkspaceCheck/2(ToolTranslation)  "<ToolTranslation>"
  ValidTrue/1 -> SafetyStatusBus/13
  StateSelect/3 -> BaseLimitChecks/1(BaseTwist)  "<BaseTwist>"
  StateSelect/2 -> JointChecks/2(ArmJointVel)  "<ArmJointVel>"
  StateSelect/1 -> JointChecks/1(ArmJointPos), WorkspaceCheck/1(ArmJointPos)  "<ArmJointPos>"
  RobotState/1 -> StateSelect/1, StalenessCheck/1(RobotState)
  WorkspaceCheck/1(Workspace) -> FlagVector/4, SafetyStatusBus/6
  StalenessCheck/2(StalePlan) -> FlagVector/8, SafetyStatusBus/10
  CausePriority/1(Cause) -> EStopLatch/2(Cause)

== system homeMobileManipulator/Perception/CaptureSchedule ==
  PlannerMode : Inport
  WristCapture : Inport  Port=2
  CaptureOr : Logic  Operator=OR  Inputs=4  AllPortsSameDT=off  OutDataTypeStr=boolean
  GroundingWindow : simulink/Logic and Bit Operations/Compare To Constant  Description=|  relop===  const=cfg.sup.pl.GROUND  OutDataTypeStr=boolean
      | THE CAPTURE GATE. True while the planner is grounding, and that is the only time the camera rig has a reader.
      | 
      | WHY THE PHASE AND NOT A WINDOW FROM t = 0. The operator app starts a run with nothing submitted, on purpose, and the instruction is typed while the apartment is already on screen - so grounding happens at an arbitrary time. A window keyed to the start of the run would answer every interactive task from a frame tens of seconds old, and hmmGroundingService would refuse it as Stale. The unattended run, whose instruction is present at t = 0, is the special case, not the general one.
      | 
      | See cfg.camera.captureWindow.
  LiveViewEnable : Constant  Value=cfg.camera.liveView  OutDataTypeStr=boolean
  LiveViewGate : Logic  AllPortsSameDT=off  OutDataTypeStr=boolean
  LiveViewPulse : DiscretePulseGenerator  PulseType=Time based  Period=cfg.camera.livePeriod  PulseWidth=100*cfg.rates.perception/cfg.camera.livePeriod
  LiveViewPulseOn : simulink/Logic and Bit Operations/Compare To Zero  relop=>  OutDataTypeStr=boolean
  StartupCapture : simulink/Logic and Bit Operations/Interval Test  Description=Opens the camera rig once early in every run (CaptureOr u4), inside cfg.camera.startupCapture, so the operator console has a picture before grounding. Not at t = 0: Unreal's auto-exposure starts dark. See LiveViewTap.  IntervalClosedRight=on  uplimit=cfg.camera.startupCapture(2)  IntervalClosedLeft=on  lowlimit=cfg.camera.startupCapture(1)  OutDataTypeStr=boolean
  StartupClock : DigitalClock  Description=Model time at the supervisor rate, for StartupCapture.  SampleTime=cfg.rates.supervisor
  LiveViewOn : Outport
  StartupOn : Outport  Port=2
  CaptureEnable : Outport  Port=3
  wires:
  StartupCapture/1 -> CaptureOr/4, StartupOn/1
  LiveViewEnable/1 -> LiveViewOn/1, LiveViewGate/2
  PlannerMode/1 -> GroundingWindow/1
  StartupClock/1 -> StartupCapture/1
  GroundingWindow/1 -> CaptureOr/1  "CaptureEnable"
  LiveViewPulseOn/1 -> LiveViewGate/1
  WristCapture/1 -> CaptureOr/2
  LiveViewGate/1 -> CaptureOr/3  "LiveViewGate"
  LiveViewPulse/1 -> LiveViewPulseOn/1
  CaptureOr/1 -> CaptureEnable/1
